simulink library "Lib_Piccolo"  (R2018b)
settings: Solver=VariableStepAuto  StartTime=0.0  StopTime=10.0  RelTol=1e-3
values from neighbouring files (symbols this model uses):
  AccelErrInt2Brakes = 0.15    [SimulationControlConfig16P.m]    (also in SimulationControlConfig16P_LEGACY.m; SimulationControlConfigTAILLESS.m = 0.2; SimulationControlConfigUTAIL.m = 0.2)
  AileronMax = 25    [SimulationControlConfig16P.m]    (also in SimulationControlConfig16P_LEGACY.m; SimulationControlConfigTAILLESS.m; SimulationControlConfigUTAIL.m)
  AileronPower = 0.00268    [SimulationControlConfig16P.m]    (also in SimulationControlConfig16P_LEGACY.m; SimulationControlConfigTAILLESS.m; SimulationControlConfigUTAIL.m)
  AileronSurfaceMax = 45    [SimulationControlConfig16P.m]    (also in SimulationControlConfig16P_LEGACY.m)
  AileronTrim = 0    [SimulationControlConfig16P.m]    (also in SimulationControlConfig16P_LEGACY.m; SimulationControlConfigTAILLESS.m; SimulationControlConfigUTAIL.m)
  Alt = 1000 + TerrainHeight    [SimulationStateConfig.m]
  AltCruise_m = testPlans(testIndx).terrainElevation * 0.3048 + 200    [SimulationControlConfig16P.m]    (also in SimulationControlConfigTAILLESS.m = 1083; SimulationControlConfigUTAIL.m = testPlans(testIndx).terrainElevation * 0.3048 + 152)
  AltitudeRate2PitchCmdIntegratorInit = 0.1    [SimulationControlPre.m]
  AltMax = 10000    [SimulationControlConfig16P.m]    (also in SimulationControlConfig16P_LEGACY.m; SimulationControlConfigTAILLESS.m; SimulationControlConfigUTAIL.m)
  AltMaxAccel = 1.25    [SimulationControlConfig16P.m]    (also in SimulationControlConfig16P_LEGACY.m = 0.9; SimulationControlConfigTAILLESS.m = 1.7; SimulationControlConfigUTAIL.m = 2)
  AltMin = 0    [SimulationControlConfig16P.m]    (also in SimulationControlConfig16P_LEGACY.m; SimulationControlConfigTAILLESS.m; SimulationControlConfigUTAIL.m)
  AltRateCmd2Pitch = 0.50    (= 0.5)    [SimulationControlConfig16P.m]    (also in SimulationControlConfig16P_LEGACY.m = 0.6; SimulationControlConfigTAILLESS.m = 0.2; SimulationControlConfigUTAIL.m = 0.3)
  AltRateError2Pitch = 0.40    (= 0.4)    [SimulationControlConfig16P.m]    (also in SimulationControlConfig16P_LEGACY.m; SimulationControlConfigTAILLESS.m = 0.55; SimulationControlConfigUTAIL.m = 0.55)
  AltRateErrorInt2Pitch = 0.50    (= 0.5)    [SimulationControlConfig16P.m]    (also in SimulationControlConfig16P_LEGACY.m = 0.45; SimulationControlConfigTAILLESS.m; SimulationControlConfigUTAIL.m = 0.75)
  AltRateLpfCutOff = 3    [SimulationControlConfig16P.m]    (also in SimulationControlConfig16P_LEGACY.m; SimulationControlConfigTAILLESS.m = 2; SimulationControlConfigUTAIL.m = 2)
  AutoNosegear2Rudder = 26    [SimulationControlConfig16P.m]    (also in SimulationControlConfig16P_LEGACY.m; SimulationControlConfigTAILLESS.m = 25.2; SimulationControlConfigUTAIL.m = 14)
  b = 5.54    [SimulationControlConfig16P.m]    (also in SimulationControlConfig16P_LEGACY.m; SimulationControlConfigTAILLESS.m = 2.37; SimulationControlConfigUTAIL.m = 2.37)
  Bank2AileronIntegratorInit = 0    [SimulationControlPre.m]
  BankMax_User = BankMax_User/180*pi    (= 0.523598775598)    [SimulationControlConfig16P.m]    (also in SimulationControlConfig16P_LEGACY.m; SimulationControlConfigTAILLESS.m = 0.610865238198; SimulationControlConfigUTAIL.m = 0.628318530718)
  baseLegFlaps = 20    [SimulationControlConfig16P.m]    (also in SimulationControlConfig16P_LEGACY.m = 0; SimulationControlConfigTAILLESS.m = 15; SimulationControlConfigUTAIL.m = 10)
  C = GeneticOpt.C    [SimulationCostFunction.m]
  c = Sw/b    (= 0.841696750903)    [SimulationControlConfig16P.m]    (also in SimulationControlConfig16P_LEGACY.m; SimulationControlConfigTAILLESS.m = 0.354008438819; SimulationControlConfigUTAIL.m = 0.354008438819)
  cell2WheelFactorMG = 5.98    [SimulationSensorConfig16P_LEGACY.m]
  cell2WheelFactorNG = 1    [SimulationSensorConfig16P_LEGACY.m]
  cellSatMaxMG = 15000    [SimulationSensorConfig16P.m]    (also in SimulationSensorConfig16P_LEGACY.m; SimulationSensorConfigTAILLESS7P.m; SimulationSensorConfigUTAIL7P.m)
  cellSatMaxNG = 1000    [SimulationSensorConfig16P.m]    (also in SimulationSensorConfig16P_LEGACY.m; SimulationSensorConfigTAILLESS7P.m; SimulationSensorConfigUTAIL7P.m)
  cellSatMinMG = -15000    [SimulationSensorConfig16P.m]    (also in SimulationSensorConfig16P_LEGACY.m; SimulationSensorConfigTAILLESS7P.m; SimulationSensorConfigUTAIL7P.m)
  cellSatMinNG = -1000    [SimulationSensorConfig16P.m]    (also in SimulationSensorConfig16P_LEGACY.m; SimulationSensorConfigTAILLESS7P.m; SimulationSensorConfigUTAIL7P.m)
  CL_Limit = CL_Max    (= 0.54)    [SimulationControlConfig16P.m]    (also in SimulationControlConfig16P_LEGACY.m; SimulationControlConfigTAILLESS.m; SimulationControlConfigUTAIL.m = 0.53)
  CL_Max = 0.54    [SimulationControlConfig16P.m]    (also in SimulationControlConfig16P_LEGACY.m; SimulationControlConfigTAILLESS.m; SimulationControlConfigUTAIL.m = 0.53)
  CL_Max_Nom = 0.465    [SimulationControlConfig16P.m]    (also in SimulationControlConfig16P_LEGACY.m; SimulationControlConfigTAILLESS.m = 0.39; SimulationControlConfigUTAIL.m)
  CL_Min = 0    [SimulationControlConfig16P.m]    (also in SimulationControlConfig16P_LEGACY.m; SimulationControlConfigTAILLESS.m; SimulationControlConfigUTAIL.m)
  ClimbMaxFraction = 0.35    [SimulationControlConfig16P.m]    (also in SimulationControlConfig16P_LEGACY.m = 0.24; SimulationControlConfigTAILLESS.m = 0.19; SimulationControlConfigUTAIL.m = 0.21)
  ClimboutMaxBank = 7.0    (= 7)    [SimulationControlConfig16P.m]    (also in SimulationControlConfig16P_LEGACY.m; SimulationControlConfigTAILLESS.m = 5; SimulationControlConfigUTAIL.m)
  ClimboutTimer = 7.0    (= 7)    [SimulationControlConfig16P.m]    (also in SimulationControlConfig16P_LEGACY.m; SimulationControlConfigTAILLESS.m; SimulationControlConfigUTAIL.m)
  dCl_per_dFlap = 0.005581818    [SimulationControlConfig16P.m]    (also in SimulationControlConfig16P_LEGACY.m = 0; SimulationControlConfigTAILLESS.m = 0; SimulationControlConfigUTAIL.m = 0)
  DecelerationCmd = 3.1    [SimulationControlConfig16P.m]    (also in SimulationControlConfig16P_LEGACY.m; SimulationControlConfigTAILLESS.m = 0.1; SimulationControlConfigUTAIL.m = 0.1)
  DeRotateLogicEndTimer = abs((NoseDownLimit_Deg-1)/DeRotateRamp_Dps)    [SimulationControlConfig16P.m]    (also in SimulationControlConfig16P_LEGACY.m; SimulationControlConfigTAILLESS.m; SimulationControlConfigUTAIL.m)
  DeRotateLogicHoldNoseUpTimer = 0.1    [SimulationControlConfig16P.m]    (also in SimulationControlConfig16P_LEGACY.m; SimulationControlConfigTAILLESS.m; SimulationControlConfigUTAIL.m)
  DeRotateLogicTimerTimeout = 2    [SimulationControlConfig16P.m]    (also in SimulationControlConfig16P_LEGACY.m; SimulationControlConfigTAILLESS.m; SimulationControlConfigUTAIL.m)
  DeRotateLowerCmdSaturation = 0    [SimulationControlConfig16P.m]    (also in SimulationControlConfig16P_LEGACY.m; SimulationControlConfigTAILLESS.m; SimulationControlConfigUTAIL.m)
  DeRotateRamp_Dps = 3    [SimulationControlConfig16P.m]    (also in SimulationControlConfig16P_LEGACY.m; SimulationControlConfigTAILLESS.m = 8; SimulationControlConfigUTAIL.m = 8)
  DeRotateUpperCmdSaturation = 7    [SimulationControlConfig16P.m]    (also in SimulationControlConfig16P_LEGACY.m; SimulationControlConfigTAILLESS.m; SimulationControlConfigUTAIL.m)
  DescentMaxFraction = 0.22    [SimulationControlConfig16P.m]    (also in SimulationControlConfig16P_LEGACY.m = 0.2; SimulationControlConfigTAILLESS.m = 0.17; SimulationControlConfigUTAIL.m = 0.17)
  DesktopSimTerrainOffset_m = 0.406    [SimulationAircraftConfig.m]
  downwindFlaps = 0    [SimulationControlConfig16P.m]    (also in SimulationControlConfig16P_LEGACY.m; SimulationControlConfigTAILLESS.m; SimulationControlConfigUTAIL.m)
  DP_init = 0.5*1.225*V_init^2    [SimulationControlConfig16P.m]    (also in SimulationControlConfig16P_LEGACY.m; SimulationControlConfigTAILLESS.m; SimulationControlConfigUTAIL.m)
  dscNoiseMG = 1    [SimulationSensorConfig16P_LEGACY.m]
  dscNoiseNG = 0.25    [SimulationSensorConfig16P_LEGACY.m]
  DSCnumBits = 24    [SimulationSensorConfig16P.m]    (also in SimulationSensorConfig16P_LEGACY.m; SimulationSensorConfigTAILLESS7P.m; SimulationSensorConfigUTAIL7P.m)
  DSCRangeMaxMG = 15000    [SimulationSensorConfig16P.m]    (also in SimulationSensorConfig16P_LEGACY.m; SimulationSensorConfigTAILLESS7P.m; SimulationSensorConfigUTAIL7P.m)
  DSCRangeMaxNG = 1000    [SimulationSensorConfig16P.m]    (also in SimulationSensorConfig16P_LEGACY.m; SimulationSensorConfigTAILLESS7P.m; SimulationSensorConfigUTAIL7P.m)
  DSCRangeMinMG = -15000    [SimulationSensorConfig16P.m]    (also in SimulationSensorConfig16P_LEGACY.m; SimulationSensorConfigTAILLESS7P.m; SimulationSensorConfigUTAIL7P.m)
  DSCRangeMinNG = -1000    [SimulationSensorConfig16P.m]    (also in SimulationSensorConfig16P_LEGACY.m; SimulationSensorConfigTAILLESS7P.m; SimulationSensorConfigUTAIL7P.m)
  dt = DLLSim.dt    [SimulationTimeStep.m]    (also in SimulationTrim.m = 0.02)
  EarlyTouchdownThreshold = 3.0    (= 3)    [SimulationControlConfig16P.m]    (also in SimulationControlConfig16P_LEGACY.m; SimulationControlConfigTAILLESS.m = 2.2; SimulationControlConfigUTAIL.m = 2.5)
  ElevatorDeflectionRate = 15    [SimulationControlConfig16P.m]    (also in SimulationControlConfig16P_LEGACY.m = 12; SimulationControlConfigTAILLESS.m = 10; SimulationControlConfigUTAIL.m = 12)
  ElevatorMax = 25    [SimulationControlConfig16P.m]    (also in SimulationControlConfig16P_LEGACY.m; SimulationControlConfigTAILLESS.m; SimulationControlConfigUTAIL.m)
  ElevatorPower = -0.002209    [SimulationControlConfig16P.m]    (also in SimulationControlConfig16P_LEGACY.m; SimulationControlConfigTAILLESS.m = -0.002956; SimulationControlConfigUTAIL.m = -0.00205983)
  ElevatorTrim = -3.5    [SimulationControlConfig16P.m]    (also in SimulationControlConfig16P_LEGACY.m; SimulationControlConfigTAILLESS.m = -6; SimulationControlConfigUTAIL.m = -8)
  elevonBias = 0    [SimulationControlConfig16P.m]    (also in SimulationControlConfig16P_LEGACY.m; SimulationControlConfigTAILLESS.m; SimulationControlConfigUTAIL.m)
  Enable_TAS_Protection = 0    [SimulationControlConfig16P.m]    (also in SimulationControlConfig16P_LEGACY.m; SimulationControlConfigTAILLESS.m; SimulationControlConfigUTAIL.m)
  EnableCrossTrackAbort = 1    [SimulationControlConfig16P.m]    (also in SimulationControlConfigTAILLESS.m; SimulationControlConfigUTAIL.m)
  EnergyBandwidth = 0.02    [SimulationControlConfig16P.m]    (also in SimulationControlConfig16P_LEGACY.m; SimulationControlConfigTAILLESS.m = 0.06; SimulationControlConfigUTAIL.m = 0.06)
  EngineLhFuelCut = 0    [SimulationAircraftConfig.m]
  EngineRhFuelCut = 0    [SimulationAircraftConfig.m]
  FastThrottleRate = 0.075    [SimulationControlConfig16P.m]    (also in SimulationControlConfig16P_LEGACY.m = 0.05; SimulationControlConfigTAILLESS.m = 0.1; SimulationControlConfigUTAIL.m = 0.1)
  FilterWarmUpTime = 2    [SimulationSensorConfig16P.m]    (also in SimulationSensorConfig16P_LEGACY.m; SimulationSensorConfigTAILLESS7P.m; SimulationSensorConfigUTAIL7P.m)
  finalApproachFlaps = 20    [SimulationControlConfig16P.m]    (also in SimulationControlConfig16P_LEGACY.m = 0; SimulationControlConfigTAILLESS.m = 22; SimulationControlConfigUTAIL.m = 10)
  FinalDescentSlope_Deg = testPlans(testIndx).descentSlope    [SimulationControlConfig16P.m]    (also in SimulationControlConfig16P_LEGACY.m; SimulationControlConfigTAILLESS.m; SimulationControlConfigUTAIL.m)
  flapMax = 0    [SimulationControlConfig16P.m]    (also in SimulationControlConfig16P_LEGACY.m; SimulationControlConfigTAILLESS.m; SimulationControlConfigUTAIL.m)
  flapRate = 7.5    [SimulationControlConfig16P.m]    (also in SimulationControlConfig16P_LEGACY.m; SimulationControlConfigTAILLESS.m = 6.6; SimulationControlConfigUTAIL.m)
  FlareHeight = 5    [SimulationControlConfig16P.m]    (also in SimulationControlConfig16P_LEGACY.m = 4.8; SimulationControlConfigTAILLESS.m = 2.5; SimulationControlConfigUTAIL.m = 2)
  FlareVerticalRate_mps = -0.4    [SimulationControlConfig16P.m]    (also in SimulationControlConfig16P_LEGACY.m = -0.5; SimulationControlConfigTAILLESS.m = -0.15; SimulationControlConfigUTAIL.m = -0.15)
  Fp_Aileron = 0.55*2*pi*RollRateLpfCutoff*dt    [SimulationControlConfig16P.m]    (also in SimulationControlConfig16P_LEGACY.m; SimulationControlConfigTAILLESS.m; SimulationControlConfigUTAIL.m)
  Fp_Alt = 0.55*AltBandwidth    (= 0.099)    [SimulationControlConfig16P.m]    (also in SimulationControlConfig16P_LEGACY.m; SimulationControlConfigTAILLESS.m = 0.587477826221; SimulationControlConfigUTAIL.m = 0.69115038379)
  Fp_AltRate = 0.55*2*pi*AltRateLpfCutOff*dt    [SimulationControlConfig16P.m]    (also in SimulationControlConfig16P_LEGACY.m; SimulationControlConfigTAILLESS.m; SimulationControlConfigUTAIL.m)
  Fp_Elevator = 0.55*2*pi*PitchRateLpfCutoff*dt    [SimulationControlConfig16P.m]    (also in SimulationControlConfig16P_LEGACY.m; SimulationControlConfigTAILLESS.m; SimulationControlConfigUTAIL.m)
  Fp_Energy = 0.55*2*pi*EnergyBandwidth    (= 0.069115038379)    [SimulationControlConfig16P.m]    (also in SimulationControlConfig16P_LEGACY.m; SimulationControlConfigTAILLESS.m = 0.207345115137; SimulationControlConfigUTAIL.m = 0.207345115137)
  Fp_Energy2 = 0.55*2*pi*EnergyBandwidth*dt    [SimulationControlConfig16P.m]    (also in SimulationControlConfig16P_LEGACY.m; SimulationControlConfigTAILLESS.m; SimulationControlConfigUTAIL.m)
  Fp_Pitch = 0.55*2*pi*PitchBandwidth    (= 2.76460153516)    [SimulationControlConfig16P.m]    (also in SimulationControlConfig16P_LEGACY.m = 3.11017672705; SimulationControlConfigTAILLESS.m = 3.80132711084; SimulationControlConfigUTAIL.m = 2.41902634326)
  Fp_Pitch_2 = 0.55*2*pi*PitchBandwidth*dt    [SimulationControlConfig16P.m]    (also in SimulationControlConfig16P_LEGACY.m; SimulationControlConfigTAILLESS.m; SimulationControlConfigUTAIL.m)
  Fp_Roll = RollBandwidth^2    (= 1)    [SimulationControlConfig16P.m]    (also in SimulationControlConfig16P_LEGACY.m = 1.44; SimulationControlConfigTAILLESS.m; SimulationControlConfigUTAIL.m)
  Fp_Rudder = 0.55*2*pi*YawRateLpfCutoff*dt    [SimulationControlConfig16P.m]    (also in SimulationControlConfig16P_LEGACY.m; SimulationControlConfigTAILLESS.m; SimulationControlConfigUTAIL.m)
  Fp_TAS = 0.55*2*pi*TASBandwidth    (= 0.103672557568)    [SimulationControlConfig16P.m]    (also in SimulationControlConfig16P_LEGACY.m; SimulationControlConfigTAILLESS.m = 0.172787595947; SimulationControlConfigUTAIL.m = 0.172787595947)
  Fp_TAS_Filter = 2*pi*TasLpfCutoff*dt    [SimulationControlConfig16P.m]    (also in SimulationControlConfig16P_LEGACY.m; SimulationControlConfigTAILLESS.m; SimulationControlConfigUTAIL.m)
  Fp_Turn = 0.55*2*pi*TurnErrLPFcutoff    (= 0.0345575191895)    [SimulationControlConfig16P.m]    (also in SimulationControlConfig16P_LEGACY.m; SimulationControlConfigTAILLESS.m = 0.172787595947; SimulationControlConfigUTAIL.m = 0.172787595947)
  Fp_TurnDerr = 0.55*2*pi*TurnDerivativeLPFcutoff    (= 0.0345575191895)    [SimulationControlConfig16P.m]    (also in SimulationControlConfig16P_LEGACY.m; SimulationControlConfigTAILLESS.m = 0.172787595947; SimulationControlConfigUTAIL.m = 0.172787595947)
  FTV = 3    [SimulationAircraftConfig.m]
  ftvStaticPositionError = 1/1.18    (= 0.847457627119)    [SimulationSensorConfig16P.m]    (also in SimulationSensorConfig16P_LEGACY.m; SimulationSensorConfigTAILLESS7P.m = 1; SimulationSensorConfigUTAIL7P.m = 1)
  g = 9.81    [SimulationStateConfig.m]
  GustSpd_Kts = testPlans(testIndx).gustSpd    [SimulationStateConfig.m]
  GustTriggerVal = testPlans(testIndx).gustTriggerVal    [SimulationStateConfig.m]
  HeadingErr2TurnRate = 0.5    [SimulationControlConfig16P.m]    (also in SimulationControlConfig16P_LEGACY.m; SimulationControlConfigTAILLESS.m; SimulationControlConfigUTAIL.m)
  HeadingErrDer2TurnRate = 0.3    [SimulationControlConfig16P.m]    (also in SimulationControlConfig16P_LEGACY.m; SimulationControlConfigTAILLESS.m; SimulationControlConfigUTAIL.m)
  IASbounce = IASstall*0.8    [SimulationControlPre.m]
  IAScruiseCMD = sqrt(2*m*9.81/(1.225*Sw*CL_cruise))    [SimulationControlConfig16P.m]    (also in SimulationControlConfig16P_LEGACY.m; SimulationControlConfigTAILLESS.m; SimulationControlConfigUTAIL.m)
  IASfinalCMD = 1.12 * IASmin    [SimulationControlConfig16P.m]    (also in SimulationControlConfig16P_LEGACY.m = 1.10 * IASmin; SimulationControlConfigTAILLESS.m = 1.10 * IASmin; SimulationControlConfigUTAIL.m = 1.15 * IASmin)
  IASflareCMD = IASstall    [SimulationControlConfig16P.m]    (also in SimulationControlConfig16P_LEGACY.m; SimulationControlConfigTAILLESS.m; SimulationControlConfigUTAIL.m)
  IASmax = 64    [SimulationControlConfig16P.m]    (also in SimulationControlConfig16P_LEGACY.m = 46; SimulationControlConfigTAILLESS.m = 38.58; SimulationControlConfigUTAIL.m = 35)
  IASmin = sqrt(2*m*9.81/(1.225*Sw*0.9*CL_Max_Nom))    [SimulationControlConfig16P.m]    (also in SimulationControlConfig16P_LEGACY.m; SimulationControlConfigTAILLESS.m; SimulationControlConfigUTAIL.m)
  IASshortCMD = IASstall    [SimulationControlConfig16P.m]    (also in SimulationControlConfig16P_LEGACY.m; SimulationControlConfigTAILLESS.m; SimulationControlConfigUTAIL.m)
  IASstall = sqrt(2*m*9.81/(1.225*Sw*CL_Max))    [SimulationControlConfig16P.m]    (also in SimulationControlConfig16P_LEGACY.m; SimulationControlConfigTAILLESS.m; SimulationControlConfigUTAIL.m)
  inFlight = 1    [SimulationControlConfig16P.m]    (also in SimulationControlConfigTAILLESS.m; SimulationControlConfigUTAIL.m)
  JetCatOffset = 5    [SimulationControlConfig16P.m]    (also in SimulationControlConfig16P_LEGACY.m)
  LaunchRollingElevator = -1.5    [SimulationControlConfig16P.m]    (also in SimulationControlConfig16P_LEGACY.m; SimulationControlConfigTAILLESS.m = 1; SimulationControlConfigUTAIL.m = 1)
  ldg_NosegearMax = 10    [SimulationControlConfig16P.m]    (also in SimulationControlConfig16P_LEGACY.m; SimulationControlConfigTAILLESS.m; SimulationControlConfigUTAIL.m)
  ldg_TrackVyErrInt2Nosegear = 0.1250    (= 0.125)    [SimulationControlConfig16P.m]    (also in SimulationControlConfig16P_LEGACY.m; SimulationControlConfigTAILLESS.m = 0.00714285714286; SimulationControlConfigUTAIL.m = 0.00714285714286)
  ldg_TrackVyErrPro2Nosegear = 0.35    [SimulationControlConfig16P.m]    (also in SimulationControlConfig16P_LEGACY.m; SimulationControlConfigTAILLESS.m = 0.0546666666667; SimulationControlConfigUTAIL.m = 0.0546666666667)
  ldg_TrackY2Vy = 0.07    [SimulationControlConfig16P.m]    (also in SimulationControlConfig16P_LEGACY.m; SimulationControlConfigTAILLESS.m = 0.17; SimulationControlConfigUTAIL.m = 0.17)
  ldg_Vy2NosegearScalingPower = 1.075    [SimulationControlConfig16P.m]    (also in SimulationControlConfig16P_LEGACY.m; SimulationControlConfigTAILLESS.m = 0.6; SimulationControlConfigUTAIL.m = 0.5)
  ldg_Y2VyScalingPower = 0.175    [SimulationControlConfig16P.m]    (also in SimulationControlConfig16P_LEGACY.m; SimulationControlConfigTAILLESS.m = 0; SimulationControlConfigUTAIL.m = 0)
  ldg_YawRate2Nosegear = 0.175    [SimulationControlConfig16P.m]    (also in SimulationControlConfig16P_LEGACY.m; SimulationControlConfigTAILLESS.m = 0.065; SimulationControlConfigUTAIL.m = 0.065)
  LiftSlope = 0.064285    [SimulationControlConfig16P.m]    (also in SimulationControlConfig16P_LEGACY.m; SimulationControlConfigTAILLESS.m = 0.058631; SimulationControlConfigUTAIL.m)
  LPFaileronInit = 0    [SimulationControlPre.m]
  LPFclestInit = 0    [SimulationControlPre.m]
  LPFenergyFFInit = 0    [SimulationControlPre.m]
  LPFtasInit = V_init + 2    [SimulationControlPre.m]
  LPFthrottleInit = ThrottleTrim    [SimulationControlPre.m]
  LPFturnErrInit = 0    [SimulationControlPre.m]
  ... (+115 more)
undefined symbols (not defined in the file or in its folder): abortFlag, alphaHPF, apmDelay, BRWNOUT, CRAWOR, CRAWUR, DiscIntNeverNeededParam, DLLSim, DLLSimStep, ECOMOR, ECOMUR, Fp_Tas, GustTrigger_HeightAgl_m, IPSTAT, LCINTEG, Ldg_Persist_Time, LOWER_FLAGS, MSG_ENABLE, NoiseStd, OLDVAL, OVERRIDE_ENABLE, OVERRIDE_VALUE, REBOOT, reversionEnable, revIASMax, revIASMin, revPitchMax, revPitchMin, revPitchRateMax, revRollMax, revRollRateMax, SAMPLE, SCALON, SensorModel, sigbuilder_block, Sim_Vx, Sim_Vy, Sim_Vz, Sim_Xpos, Sim_Ypos, Sim_Zpos, SYSOR, SYSUR, TARE, TEMPOR, TEMPUR, testIndx, testPlan, testPlans, Trim_piccoloInCmd, Trim_REFSI_FD_IN_nmodeCgShifterCmd_Ft, Trim_REFSI_FD_IN_nmodeFlapLhIBCmd_Deg, Trim_REFSI_FD_IN_nmodeFlapLhOBCmd_Deg, Trim_REFSI_FD_IN_nmodeFlapRhIBCmd_Deg, Trim_REFSI_FD_IN_nmodeFlapRhOBCmd_Deg, Trim_REFSI_FD_IN_nmodeSlatLhCmd_Deg, Trim_REFSI_FD_IN_nmodeSlatRhCmd_Deg, Trim_REFSI_FD_IN_nmodeSplrLhInbdCmd_Deg, Trim_REFSI_FD_IN_nmodeSplrLhOutbdCmd_Deg ... (+5)
libraries: simulink x866, aerolibconvert2 x60, $bdroot x52, aerolibatmos2 x5, dspswit3 x5, simulink_extras x4, dsparch4 x2, Lib_Piccolo_Alt x2, eeGeneralControl x1, dspindex x1
(part 4 of 44)

== system Lib_Piccolo/IAS Min Calc ==
  Compare To Constant : simulink/Logic and Bit Operations/Compare To Constant  relop=<  const=10  OutDataTypeStr=boolean
  Constant : Constant  Value=(2*m*g)
  Constant1 : Constant  Value=CL_Max
  Constant2 : Constant  Value=CL_Max_Nom
  Constant3 : Constant  Value=(2*m*g)
  Divide : Product  Inputs=*/
  Divide1 : Product  Inputs=*/
  Gain : Gain  Gain=dCl_per_dFlap
  Gain1 : Gain  Gain=1.225*Sw*0.9
  Gain2 : Gain  Gain=1.225*Sw
  Sqrt : Sqrt  SaturateOnIntegerOverflow=on
  Sqrt1 : Sqrt  SaturateOnIntegerOverflow=on
  Sum : Sum  Inputs=|++
  Sum1 : Sum  Inputs=++|
  Switch : Switch  Criteria=u2 > Threshold  Threshold=0.5
  Terminator : Terminator
  IASmin : Outport
  tag scope: IASmin=global, IASstall=global
  wires:
  Sqrt/1 -> Switch/1, [IASmin]  "Sim.IASmin"
  Constant/1 -> Divide/1
  Constant2/1 -> Sum/1
  [flapCmd] -> Gain/1
  Gain/1 -> Sum1/1, Sum/2
  Sum/1 -> Gain1/1
  Gain1/1 -> Divide/2
  Divide/1 -> Sqrt/1
  Constant1/1 -> Sum1/2
  Sum1/1 -> Gain2/1
  Gain2/1 -> Divide1/2
  Constant3/1 -> Divide1/1
  Divide1/1 -> Sqrt1/1
  Sqrt1/1 -> Switch/3, Terminator/1, [IASstall]  "Sim.IASstall"
  Switch/1 -> IASmin/1  "Sim.IASminAP"
  [Pic_AP_Mode] -> Compare To Constant/1
  Compare To Constant/1 -> Switch/2

== system Lib_Piccolo/LDG TAS Cmd ==
  note: Check if in Short Final
  note: Check if in Flare
  Feedback Bus : Inport
  Bus Selector : BusSelector  OutputSignals=apMode
  Bus Selector1 : BusSelector  OutputSignals=apMode
  CAS2TAS : Subsystem
  Compare To Constant1 : simulink/Logic and Bit Operations/Compare To Constant  relop=>=  const=10  OutDataTypeStr=boolean
  Compare To Constant4 : simulink/Logic and Bit Operations/Compare To Constant  relop=>=  const=9  OutDataTypeStr=boolean
  Constant : Constant  Value=IASmax
  Constant2 : Constant  Value=IASshortCMD+testPlans(testIndx).speedOffset
  Constant3 : Constant  Value=IASfinalCMD+testPlans(testIndx).speedOffset
  Constant4 : Constant  Value=IASflareCMD
  IAS Min Calc : $bdroot/IAS Min Calc  SystemSampleTime=-1
  Multiply : Product
  NOT : Logic  Operator=NOT  IconShape=distinctive  AllPortsSameDT=off  OutDataTypeStr=boolean
  NOT1 : Logic  Operator=NOT  IconShape=distinctive  AllPortsSameDT=off  OutDataTypeStr=boolean
  Saturation Dynamic : simulink/Discontinuities/Saturation Dynamic  OutMin=[]  OutMax=[]  OutDataTypeStr=Inherit: Same as second input  OutDataType=fixdt(1, 16)  OutScaling=2^-10  DoSatur=off
  Switch1 : Switch  Criteria=u2 > Threshold
  Switch2 : Switch  Criteria=u2 > Threshold
  Sim.TAScmd : Outport
  tag scope: Sim_TAScmd=global
  wires:
  CAS2TAS/1(Out1) -> Multiply/2
  Switch2/1 -> Saturation Dynamic/2
  Constant2/1 -> Switch2/3
  Constant4/1 -> Switch1/3
  Constant3/1 -> Switch2/1
  Switch1/1 -> Multiply/1  "Sim.IAScmd"
  Multiply/1 -> [Sim_TAScmd], Sim.TAScmd/1  "Sim.TAScmd"
  Compare To Constant4/1 -> NOT/1
  Bus Selector/1 -> Compare To Constant4/1  "<apMode>"
  NOT/1 -> Switch2/2
  Feedback Bus/1 -> Bus Selector1/1, Bus Selector/1, CAS2TAS/1(In1)
  Bus Selector1/1 -> Compare To Constant1/1  "<apMode>"
  Compare To Constant1/1 -> NOT1/1
  NOT1/1 -> Switch1/2
  IAS Min Calc/1 -> Saturation Dynamic/3
  Constant/1 -> Saturation Dynamic/1
  Saturation Dynamic/1 -> Switch1/1

== system Lib_Piccolo/LDG TAS Cmd No Offset ==
  note: Check if in Short Final
  note: Check if in Flare
  Feedback Bus : Inport
  Bus Selector : BusSelector  OutputSignals=apMode
  Bus Selector1 : BusSelector  OutputSignals=apMode
  CAS2TAS : Subsystem
  Compare To Constant1 : simulink/Logic and Bit Operations/Compare To Constant  relop=>=  const=10  OutDataTypeStr=boolean
  Compare To Constant4 : simulink/Logic and Bit Operations/Compare To Constant  relop=>=  const=9  OutDataTypeStr=boolean
  Constant : Constant  Value=IASmax
  Constant2 : Constant  Value=IASshortCMD
  Constant3 : Constant  Value=IASfinalCMD
  Constant4 : Constant  Value=IASflareCMD
  IAS Min Calc : $bdroot/IAS Min Calc  SystemSampleTime=-1
  Multiply : Product
  NOT : Logic  Operator=NOT  IconShape=distinctive  AllPortsSameDT=off  OutDataTypeStr=boolean
  NOT1 : Logic  Operator=NOT  IconShape=distinctive  AllPortsSameDT=off  OutDataTypeStr=boolean
  Saturation Dynamic : simulink/Discontinuities/Saturation Dynamic  OutMin=[]  OutMax=[]  OutDataTypeStr=Inherit: Same as second input  OutDataType=fixdt(1, 16)  OutScaling=2^-10  DoSatur=off
  Switch1 : Switch  Criteria=u2 > Threshold
  Switch2 : Switch  Criteria=u2 > Threshold
  Sim.TAScmd : Outport
  tag scope: Sim_TAScmd=global
  wires:
  CAS2TAS/1(Out1) -> Multiply/2
  Switch2/1 -> Saturation Dynamic/2
  Constant2/1 -> Switch2/3
  Constant4/1 -> Switch1/3
  Constant3/1 -> Switch2/1
  Switch1/1 -> Multiply/1  "Sim.IAScmd"
  Multiply/1 -> [Sim_TAScmd], Sim.TAScmd/1  "Sim.TAScmd"
  Compare To Constant4/1 -> NOT/1
  Bus Selector/1 -> Compare To Constant4/1  "<apMode>"
  NOT/1 -> Switch2/2
  Feedback Bus/1 -> Bus Selector1/1, Bus Selector/1, CAS2TAS/1(In1)
  Bus Selector1/1 -> Compare To Constant1/1  "<apMode>"
  Compare To Constant1/1 -> NOT1/1
  NOT1/1 -> Switch1/2
  IAS Min Calc/1 -> Saturation Dynamic/3
  Constant/1 -> Saturation Dynamic/1
  Saturation Dynamic/1 -> Switch1/1

== system Lib_Piccolo/Latch ==
  D : Inport
  Enable/!Rst : Inport  Port=2
  AND : Logic  IconShape=distinctive  AllPortsSameDT=off  OutDataTypeStr=boolean
  Constant : Constant
  OR : Logic  Operator=OR  IconShape=distinctive  AllPortsSameDT=off  OutDataTypeStr=boolean
  Switch : Switch  Criteria=u2 > Threshold  Threshold=0.5
  Unit Delay : UnitDelay  SampleTime=-1
  Q_Latched : Outport
  wires:
  Unit Delay/1 -> OR/2
  Switch/1 -> Q_Latched/1, Unit Delay/1
  D/1 -> Switch/3, OR/1
  OR/1 -> AND/1
  AND/1 -> Switch/2
  Enable/!Rst/1 -> AND/2
  Constant/1 -> Switch/1

== system Lib_Piccolo/Pic Airspeed Model ==
  note: $\rho = \frac{P\cdot MW}{R\cdot T}$
  note: $IAS = \sqrt{\frac{2\cdot P_{dynamic}}{\rho_0}}$
  note: $P_{dynamic} = P_{dynamic\_sensor} \cdot Correction$
  note: $P_{static} = P_{static} + P_{dynamic\_sensor} - P_{dynamic}$
  note: $TAS = \frac{IAS}{\sqrt{\frac{\rho}{\rho_0}}}$
  OAT_C : Inport
  Static_Pa : Inport  Port=2
  Dynamic_Pa : Inport  Port=3
  Constant : Constant  Value=0
  Constant1 : Constant  Value=0
  Divide{,1..3} (4 alike) : Product  Inputs=*/
  Gain : Gain  Gain=2
  Gain1 : Gain  Gain=correction
  Ideal Gas Constant : Gain  Gain=8.314463
  Kelvin Offset : Constant  Value=273.15
  MW (kg/mol) : Gain  Gain=28.9647/1000
  Max : MinMax  Function=max  Inputs=2
  Max1 : MinMax  Function=max  Inputs=2
  Sqrt : Sqrt  SaturateOnIntegerOverflow=on
  Sqrt1 : Sqrt  SaturateOnIntegerOverflow=on
  Sum : Sum  Inputs=++|
  Sum1 : Sum  Inputs=-++
  rho SL ISA : Constant  Value=1.225
  TAS : Outport
  IAS : Outport  Port=2
  Sim.PicDensity_kg/m3 : Outport  Port=3
  wires:
  OAT_C/1 -> Sum/2
  Kelvin Offset/1 -> Sum/1
  Sum/1 -> Ideal Gas Constant/1
  MW (kg/mol)/1 -> Divide/1
  Ideal Gas Constant/1 -> Divide/2
  Divide/1 -> Sim.PicDensity_kg/m3/1, Divide2/1  "IdealDensity_kg/m3"
  Gain1/1 -> Sum1/1, Gain/1  "Pdynamic"
  Gain/1 -> Divide1/1
  Divide1/1 -> Max/1
  rho SL ISA/1 -> Divide2/2, Divide1/2
  Divide2/1 -> Max1/1
  Divide3/1 -> TAS/1  "Sim.Pic_TAS"
  Sqrt/1 -> IAS/1, Divide3/1  "Sim.Pic_IAS"
  Dynamic_Pa/1 -> Sum1/2, Gain1/1  "Pdynamic_sensor"
  Sum1/1 -> MW (kg/mol)/1  "Pstatic"
  Sqrt1/1 -> Divide3/2
  Static_Pa/1 -> Sum1/3
  Max/1 -> Sqrt/1
  Constant/1 -> Max/2
  Constant1/1 -> Max1/2
  Max1/1 -> Sqrt1/1

== system Lib_Piccolo/Piccolo State Machine ==
  SimOutBus In : Inport
  In1 : Inport  Port=2
  Bus Assignment : BusAssignment  AssignedSignals=apMode
  Bus Selector : BusSelector  OutputSignals=apMode,IAS_mps,Sim_VGround
  Constant4 : Constant  Value=inFlight
  Flight State Machine : Subsystem
  Landing State Machine : Subsystem
  Switch4 : Switch  Threshold=1
  SimOutBus Out : Outport
  Out1 : Outport  Port=2
  tag scope: Pic_AP_Mode=global
  wires:
  Bus Selector/3 -> Flight State Machine/3(GroundSpeed)  "<Sim_VGround>"
  In1/1 -> Bus Assignment/1, Bus Selector/1
  Bus Assignment/1 -> Out1/1
  SimOutBus In/1 -> SimOutBus Out/1
  Constant4/1 -> Switch4/2  "inFlight"
  Bus Selector/1 -> Flight State Machine/1(<apMode>), Landing State Machine/1(<apMode>)  "<apMode>"
  Landing State Machine/1(Sim.apMode) -> Switch4/3
  Flight State Machine/1(Sim.apMode) -> Switch4/1
  Switch4/1 -> [Pic_AP_Mode], Bus Assignment/2  "Sim.apMode"
  Bus Selector/2 -> Flight State Machine/2(IAS)  "<IAS_mps>"

== system Lib_Piccolo/Piccolo State Machine FLIGHT LEGACY ==
  note: Assume maneuvers performed in 'Flying' State
  note: Moved to Vertical Track Following Guidance in Next Block
  SimOutBus In : Inport
  In1 : Inport  Port=2
  Bus Assignment : BusAssignment  AssignedSignals=apMode
  Constant : Constant  Value=4  OutDataTypeStr=uint8
  Flare Detection : Subsystem
  ShortFinal Detection : Subsystem  Commented=on
  SimOutBus Out : Outport
  Out1 : Outport  Port=2
  tag scope: Pic_AP_Mode=global
  wires:
  In1/1 -> Bus Assignment/1
  Constant/1 -> Bus Assignment/2, [Pic_AP_Mode]  "Sim.apMode"
  Bus Assignment/1 -> Out1/1
  SimOutBus In/1 -> SimOutBus Out/1

== system Lib_Piccolo/Piccolo State Machine LDG ==
  note: Moved to Vertical Track Following Guidance in Next Block
  SimOutBus In : Inport
  In1 : Inport  Port=2
  Bus Assignment : BusAssignment  AssignedSignals=apMode
  Bus Selector : BusSelector  OutputSignals=apMode
  Compare To Constant1 : simulink/Logic and Bit Operations/Compare To Constant  relop=>  const=0  OutDataTypeStr=boolean
  Constant : Constant  Value=9
  Constant1 : Constant  Value=10
  Constant2 : Constant  Value=11
  Constant3 : Constant  Value=8
  Data Type Conversion : DataTypeConversion  OutDataTypeStr=uint8
  Flare Detection : Subsystem
  FlareLatch : Subsystem
  NOT : Logic  Operator=NOT  IconShape=distinctive  AllPortsSameDT=off  OutDataTypeStr=boolean
  NOT1 : Logic  Operator=NOT  IconShape=distinctive  AllPortsSameDT=off  OutDataTypeStr=boolean
  ShortFinal Detection : Subsystem  Commented=on
  Switch{,1..3} (4 alike) : Switch  Criteria=u2 > Threshold
  SimOutBus Out : Outport
  Out1 : Outport  Port=2
  tag scope: Pic_AP_Mode=global
  wires:
  In1/1 -> Bus Assignment/1, Bus Selector/1
  [ShortFinalFlag] -> Compare To Constant1/1
  Constant/1 -> Switch/3
  Switch/1 -> Switch1/1
  Constant1/1 -> Switch1/3
  Switch1/1 -> Switch2/1
  Constant2/1 -> Switch2/3
  Switch2/1 -> Data Type Conversion/1, [Pic_AP_Mode]  "Sim.apMode"
  Bus Selector/1 -> Switch3/1  "<apMode>"
  Bus Assignment/1 -> Out1/1
  Compare To Constant1/1 -> Switch/2
  SimOutBus In/1 -> SimOutBus Out/1
  Switch3/1 -> Switch/1
  [FinalFlag] -> NOT1/1
  Constant3/1 -> Switch3/3
  NOT1/1 -> Switch3/2
  [FlareFlag] -> FlareLatch/2(FlareFlag)
  FlareLatch/1(FlareLatch) -> Switch1/2
  [Pic_AP_Mode] -> FlareLatch/1(apMode)
  NOT/1 -> Switch2/2
  [TouchdownDetectedFlag] -> NOT/1
  Data Type Conversion/1 -> Bus Assignment/2

== system Lib_Piccolo/Pitch to Elevator ==
  note: Euler to Body Conversion, Reference Signal Generation
  note: Scalar Saturation
  note: Output Filtering, Ramp & Reversion Logic
  note: Dynamic Inversion Components
  note: P I Components
  note: Damp and STIFF are non-dimentional;
      | CP has the unit of 1/deg
  PitchCmd_Euler : Inport
  Feedback Bus : Inport  Port=2
  1-K_TD : Gain  Gain=1-PitchDampingTrust
  1/ElevatorPower : Gain  Gain=1/ElevatorPower
  "1/ElevatorPower  " : Gain  Gain=1/ElevatorPower
  1st Order Reference Model : Subsystem
  Bus Selector : BusSelector  OutputSignals=Pitch_Euler_rad,Roll_Euler_rad,apMode,DynamicPressure_Pa,PitchRate_Body_radps,V_mps,zAccel_Body_mps2
  Cm/Alpha Estimation : Subsystem
  Compare To Constant : simulink/Logic and Bit Operations/Compare To Constant  relop=<=  const=2  OutDataTypeStr=boolean
  Compare To Constant1 : simulink/Logic and Bit Operations/Compare To Constant  relop===  const=11  OutDataTypeStr=uint8
  Dimensional Elevator Power : Subsystem
  Discrete-Time Integrator1 : DiscreteIntegrator  IntegratorMethod=Integration: Backward Euler  ExternalReset=level  InitialConditionSource=external  SampleTime=-1  LimitOutput=on  UpperSaturationLimit=ElevatorMax  LowerSaturationLimit=-ElevatorMax  ICPrevOutput=DiscIntNeverNeededParam  ICPrevScaledInput=DiscIntNeverNeededParam
  Divide : Product  Inputs=/*
  DynamicPLimit : Subsystem
  Elevator Ramp Logic : Subsystem
  Gain : Gain  Gain=180/pi
  Gain1 : Gain  Gain=-1
  Gain2 : Gain  Gain=pi/180
  Gain3 : Gain  Gain=-1
  KI_Pitch : Gain  Gain=PitchRateErrorInt2Accel
  K_TD : Gain  Gain=PitchDampingTrust
  K_TS : Gain  Gain=PitchStiffnessTrust
  Kp_Pitch : Gain  Gain=PitchRateError2Accel
  LPF Elevator : Subsystem
  Manual Switch : ManualSwitch  CurrentSetting=0
  Manual Switch1 : ManualSwitch  CurrentSetting=0
  NOT : Logic  Operator=NOT  IconShape=distinctive  AllPortsSameDT=off  OutDataTypeStr=boolean
  NOT1 : Logic  Operator=NOT  IconShape=distinctive  AllPortsSameDT=off  OutDataTypeStr=boolean
  OR : Logic  Operator=OR  IconShape=distinctive  AllPortsSameDT=off  OutDataTypeStr=boolean
  Pitch Moment Caused By Damping : Subsystem
  Rad2Deg : Gain  Gain=180/pi
  Reference Frame Conversion and Pitch Rate Limit Determination : Subsystem
  Saturation : Saturate  UpperLimit=ElevatorMax  LowerLimit=-ElevatorMax
  Sum : Sum  Inputs=|+-
  Sum1 : Sum  Inputs=|+--+
  Sum2 : Sum  Inputs=|++
  Sum3 : Sum  Inputs=++|
  Switch : Switch  Criteria=u2 > Threshold
  TASLimit : Subsystem
  Terminator{1..4} (4 alike) : Terminator
  Triggered Subsystem : Subsystem  TreatAsAtomicUnit=on
  Unit Delay : UnitDelay  SampleTime=-1
  constant : Constant  Value=ElevatorTrim  VectorParams1D=off
  resetCondition : Subsystem
  resetVal : Subsystem
  Elevator_Deg : Outport
  tag scope: PicElevatorOut=global, Sim_PitchCmd=global, Sim_PitchRateCmd=global
  wires:
  Compare To Constant1/1 -> OR/2
  OR/1 -> Triggered Subsystem/Trigger, NOT/1
  Compare To Constant/1 -> OR/1
  Rad2Deg/1 -> Terminator1/1  "Sim.PitchCmd"
  resetCondition/1(reset) -> Discrete-Time Integrator1/2
  Bus Selector/6 -> Reference Frame Conversion and Pitch Rate Limit Determination/4(V), TASLimit/2(<V_mps>)  "<V_mps>"
  TASLimit/1(Out1) -> Pitch Moment Caused By Damping/2(TAS)
  Bus Selector/4 -> DynamicPLimit/2(DynamicPressure_Pa)  "<DynamicPressure_Pa>"
  DynamicPLimit/1(Out1) -> Cm/Alpha Estimation/2(Q), Reference Frame Conversion and Pitch Rate Limit Determination/5(Q), Dimensional Elevator Power/1(Dynamic Pressure (Avoid Small Value))
  [Pic_AP_Mode] -> Compare To Constant1/1, Compare To Constant/1
  NOT/1 -> Switch/2
  Switch/1 -> LPF Elevator/1(Input)
  Triggered Subsystem/1(Out1) -> [Elevator_Offset]  "ElevatorOffset"
  Unit Delay/1 -> Triggered Subsystem/1(In1)
  Saturation/1 -> Unit Delay/1, Elevator_Deg/1, Manual Switch1/2  "elevOut"
  [Elevator_Offset] -> Sum1/4
  Reference Frame Conversion and Pitch Rate Limit Determination/3("Scalar ") -> 1st Order Reference Model/3("Scalar ")
  Reference Frame Conversion and Pitch Rate Limit Determination/5("PitchRateLimit_Max ") -> 1st Order Reference Model/5("PitchRateLimit_Max ")
  Sum2/1 -> Pitch Moment Caused By Damping/1(PitchRate_Body)  "Sim.Damp_TrustMix"
  1/ElevatorPower/1 -> Sum1/2, Gain1/1
  Gain2/1 -> Manual Switch/1  "REF.pitchRateCmd"
  Manual Switch/1 -> Sum/1, 1-K_TD/1
  [REFpitchRateCmd] -> Gain2/1  "REF.pitchRateCmdDps"
  Pitch Moment Caused By Damping/1(DAMP) -> 1/ElevatorPower/1
  constant/1 -> Terminator4/1  "Sim.PitchTrim"
  Discrete-Time Integrator1/1 -> Sum3/1  "Sim.KI_Pitch"
  Kp_Pitch/1 -> Sum3/2  "Sim.Kp_Pitch"
  Sum3/1 -> Sum1/1
  Divide/1 -> KI_Pitch/1, Kp_Pitch/1
  KI_Pitch/1 -> Discrete-Time Integrator1/1
  Bus Selector/3 -> 1st Order Reference Model/7(apMode), TASLimit/1(apMode), DynamicPLimit/1(apMode)  "<apMode>"
  Gain/1 -> [Sim_PitchRateCmd]  "Sim.pitchRateCmd"
  Gain1/1 -> Terminator2/1  "Sim.PitchDamp"
  Gain3/1 -> Terminator3/1  "Sim.PitchStiffness"
  "1/ElevatorPower  "/1 -> Sum1/3, Gain3/1
  Sum1/1 -> Switch/1
  Bus Selector/7 -> Cm/Alpha Estimation/1(zAccel_Body)  "<zAccel_Body_mps2>"
  Bus Selector/5 -> 1st Order Reference Model/8(PitchRate_Body), Sum/2, K_TD/1  "<PitchRate_Body_radps>"
  Bus Selector/2 -> Reference Frame Conversion and Pitch Rate Limit Determination/3(Roll_Euler)  "<Roll_Euler_rad>"
  Bus Selector/1 -> Reference Frame Conversion and Pitch Rate Limit Determination/2(Pitch_Euler)  "<Pitch_Euler_rad>"
  Feedback Bus/1 -> Bus Selector/1
  Reference Frame Conversion and Pitch Rate Limit Determination/6("PitchRateLimit_Min ") -> 1st Order Reference Model/6(" PitchRateLimit_Min ")
  Reference Frame Conversion and Pitch Rate Limit Determination/4(PitchRateCmd_Body) -> 1st Order Reference Model/4("PitchRateCmd_Body ")
  PitchCmd_Euler/1 -> [Sim_PitchCmd], Rad2Deg/1, Reference Frame Conversion and Pitch Rate Limit Determination/1(PitchCmd_Euler)
  Dimensional Elevator Power/1(CP) -> Divide/1
  Reference Frame Conversion and Pitch Rate Limit Determination/2("Pitch_Body ") -> 1st Order Reference Model/2("Pitch_Body ")
  Cm/Alpha Estimation/1(STIFF) -> K_TS/1
  K_TD/1 -> Sum2/2
  1-K_TD/1 -> Sum2/1
  1st Order Reference Model/1(PitchRateCmd_Body) -> Gain/1, Manual Switch/2
  Sum/1 -> Divide/2  "Sim.pitchRateErr"
  Reference Frame Conversion and Pitch Rate Limit Determination/1(PitchCmd_Body) -> 1st Order Reference Model/1(PitchCmd_Body)
  [ApGlobal] -> NOT1/1
  NOT1/1 -> LPF Elevator/2(Reset)
  [pilotPitch] -> LPF Elevator/3(ResetValue)  "rstVal"
  resetVal/1(resetVal) -> Discrete-Time Integrator1/3
  Manual Switch1/1 -> [PicElevatorOut]
  [REF_elevator] -> Manual Switch1/1
  Elevator Ramp Logic/1(Elevator Out) -> Switch/3, Saturation/1
  LPF Elevator/1(Output) -> Elevator Ramp Logic/1(Elevator In)  "elevLPFout"
  [Pic_AP_Mode] -> Elevator Ramp Logic/2(AP Mode)
  K_TS/1 -> "1/ElevatorPower  "/1

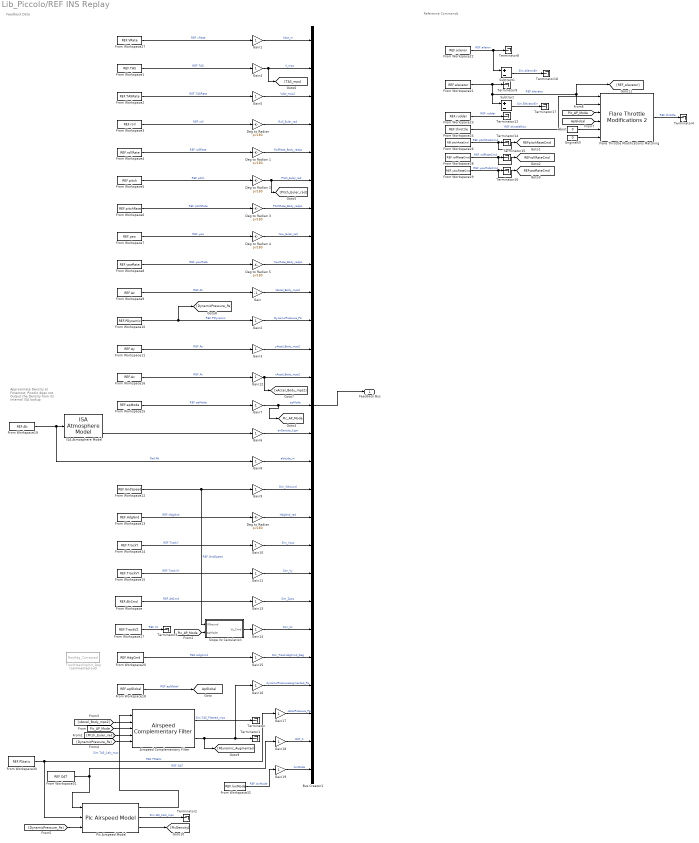
== system Lib_Piccolo/REF INS Replay ==
  note: Feedback Data
  note: Approximate Density at Foremost. Piccolo does not Output the Density from its internal ISA lookup
  note: Reference Commands
  Abort : Constant  Value=0
  Airspeed Complementary Filter : $bdroot/Airspeed Complementary Filter  SystemSampleTime=-1
  Bus Creator1 : BusCreator  Inputs=27
  Deg to Radian : Gain  Gain=pi/180
  Deg to Radian {,1..5} (6 alike) : Gain  Gain=pi/180
  EngineKill : Constant  Value=0
  Flare Throttle Modifications Matching : $bdroot/Throttle Control (Alt Mode)/Flare Throttle Modifications 2  SystemSampleTime=-1
  From Workspace : FromWorkspace  VariableName=REF.AltCmd  SampleTime=0
  From Workspace1 : FromWorkspace  VariableName=REF.TAS  SampleTime=0
  From Workspace10 : FromWorkspace  VariableName=REF.PDynamic  SampleTime=0
  From Workspace11 : FromWorkspace  VariableName=REF.Ay  SampleTime=0
  From Workspace12 : FromWorkspace  VariableName=REF.GndSpeed  SampleTime=0
  From Workspace13 : FromWorkspace  VariableName=REF.HdgGnd  SampleTime=0
  From Workspace14 : FromWorkspace  VariableName=REF.TrackY  SampleTime=0
  From Workspace15 : FromWorkspace  VariableName=REF.TrackVY  SampleTime=0
  From Workspace16 : FromWorkspace  VariableName=REF.Ax  SampleTime=0
  From Workspace17 : FromWorkspace  VariableName=REF.TrackVZ  SampleTime=0
  From Workspace18 : FromWorkspace  VariableName=REF.apGlobal  SampleTime=0
  From Workspace19 : FromWorkspace  VariableName=REF.Alt  SampleTime=0
  From Workspace2 : FromWorkspace  VariableName=REF.TASRate  SampleTime=0
  From Workspace20 : FromWorkspace  VariableName=REF.HdgCmd  SampleTime=0
  From Workspace21 : FromWorkspace  VariableName=REF.elevator  SampleTime=0
  From Workspace22 : FromWorkspace  VariableName=REF.aileron  SampleTime=0
  From Workspace23 : FromWorkspace  VariableName=REF.rudder  SampleTime=0
  From Workspace24 : FromWorkspace  VariableName=REF.throttle  SampleTime=0
  From Workspace25 : FromWorkspace  VariableName=REF.apMode  SampleTime=0
  From Workspace26 : FromWorkspace  VariableName=REF.pitchRateCmd  SampleTime=0
  From Workspace27 : FromWorkspace  VariableName=REF.VRate  SampleTime=0
  From Workspace28 : FromWorkspace  VariableName=REF.rollRateCmd  SampleTime=0
  From Workspace29 : FromWorkspace  VariableName=REF.yawRateCmd  SampleTime=0
  From Workspace3 : FromWorkspace  VariableName=REF.roll  SampleTime=0
  From Workspace30 : FromWorkspace  VariableName=REF.PStatic  SampleTime=0
  From Workspace31 : FromWorkspace  VariableName=REF.OAT  SampleTime=0
  From Workspace32 : FromWorkspace  VariableName=REF.lonMode  SampleTime=0
  From Workspace4 : FromWorkspace  VariableName=REF.rollRate  SampleTime=0
  From Workspace5 : FromWorkspace  VariableName=REF.pitch  SampleTime=0
  From Workspace6 : FromWorkspace  VariableName=REF.pitchRate  SampleTime=0
  From Workspace7 : FromWorkspace  VariableName=REF.yaw  SampleTime=0
  From Workspace8 : FromWorkspace  VariableName=REF.yawRate  SampleTime=0
  From Workspace9 : FromWorkspace  VariableName=REF.Az  SampleTime=0
  Gain : Gain  Gain=-1
  Gain{1..19} (19 alike) : Gain
  ISA Atmosphere Model : aerolibatmos2/ISA Atmosphere Model  custom=off  g=9.80665  gamma=1.4  R=287.0531  L=0.0065  h_trop=11000  h_strat=20000  rho0=1.225  P0=101325  T0=288.15  h0=0
      settings: SourceProductName=Aerospace Blockset
  Pic Airspeed Model : $bdroot/Pic Airspeed Model  correction=1
  Slope Vz Calculation : Subsystem
  Subtract : Sum  Inputs=+-
  Subtract1 : Sum  Inputs=+-
  Terminator{,1..4,8..9,12,14..18} (13 alike) : Terminator
  TrackHeadingInit_Deg : Constant  Commented=on  Value=RwyHdg_Corrected
  Feedback Bus : Outport
  tag scope: ApGlobal=global, Pic_AP_Mode=global, REFpitchRateCmd=global, REFrollRateCmd=global, REFyawRateCmd=global
  wires:
  Deg to Radian 2/1 -> [Pitch_Euler_rad], Bus Creator1/6  "Pitch_Euler_rad"
  Deg to Radian 3/1 -> Bus Creator1/7  "PitchRate_Body_radps"
  Gain/1 -> Bus Creator1/10  "zAccel_Body_mps2"
  Deg to Radian 5/1 -> Bus Creator1/9  "YawRate_Body_radps"
  Deg to Radian 4/1 -> Bus Creator1/8  "Yaw_Euler_rad"
  Bus Creator1/1 -> Feedback Bus/1
  Gain3/1 -> Bus Creator1/12  "yAccel_Body_mps2"
  Gain1/1 -> Bus Creator1/1  "hdot_m"
  Gain4/1 -> [TAS_mps], Bus Creator1/2  "V_mps"
  Gain5/1 -> Bus Creator1/3  "Vdot_mps2"
  "Deg to Radian "/1 -> Bus Creator1/4  "Roll_Euler_rad"
  Deg to Radian 1/1 -> Bus Creator1/5  "RollRate_Body_radps"
  Gain6/1 -> Bus Creator1/15  "airDensity_kgm"
  From Workspace27/1 -> Gain1/1  "REF.vRate"
  From Workspace2/1 -> Gain5/1  "REF.TASRate"
  From Workspace3/1 -> "Deg to Radian "/1  "REF.roll"
  From Workspace4/1 -> Deg to Radian 1/1  "REF.rollRate"
  From Workspace5/1 -> Deg to Radian 2/1  "REF.pitch"
  From Workspace6/1 -> Deg to Radian 3/1  "REF.pitchRate"
  From Workspace7/1 -> Deg to Radian 4/1  "REF.yaw"
  From Workspace8/1 -> Deg to Radian 5/1  "REF.yawRate"
  From Workspace9/1 -> Gain/1  "REF.Az"
  From Workspace10/1 -> [DynamicPressure_Pa], Gain2/1  "REF.PDynamic"
  From Workspace11/1 -> Gain3/1  "REF.Ay"
  ISA Atmosphere Model/4 -> Gain6/1
  From Workspace19/1 -> Gain8/1, ISA Atmosphere Model/1  "Ref.Alt"
  Gain7/1 -> [Pic_AP_Mode], Bus Creator1/14  "apMode"
  From Workspace25/1 -> Gain7/1  "REF.apMode"
  Gain8/1 -> Bus Creator1/16  "altitude_m"
  Gain9/1 -> Bus Creator1/17  "Sim_VGround"
  From Workspace12/1 -> Slope Vz Calculation/1(VGround), Gain9/1  "REF.GndSpeed"
  From Workspace13/1 -> Deg to Radian/1  "REF.HdgGnd"
  Deg to Radian/1 -> Bus Creator1/18  "HdgGnd_rad"
  From Workspace1/1 -> Gain4/1  "REF.TAS"
  From Workspace14/1 -> Gain10/1  "REF.TrackY"
  Gain10/1 -> Bus Creator1/19  "Sim_Ypos"
  From Workspace15/1 -> Gain11/1  "REF.TrackVY"
  Gain11/1 -> Bus Creator1/20  "Sim_Vy"
  From Workspace16/1 -> Gain12/1  "REF.Ax"
  Gain12/1 -> [xAccel_Body_mps2], Bus Creator1/13  "xAccel_Body_mps2"
  From Workspace/1 -> Gain13/1  "REF.AltCmd"
  Gain13/1 -> Bus Creator1/21  "Sim_Zpos"
  Gain14/1 -> Bus Creator1/22  "Sim_Vz"
  From Workspace17/1 -> Terminator3/1  "REF.Vz"
  From Workspace18/1 -> [ApGlobal]  "REF.apGlobal"
  Gain15/1 -> Bus Creator1/23  "Sim_TrackHdgCmd_Deg"
  From Workspace20/1 -> Gain15/1  "REF.HdgCmd"
  [Pic_AP_Mode] -> Airspeed Complementary Filter/3
  [Pitch_Euler_rad] -> Airspeed Complementary Filter/4
  [xAccel_Body_mps2] -> Airspeed Complementary Filter/2
  Airspeed Complementary Filter/1 -> Terminator/1  "Sim.TAS_Filtered_mps"
  [DynamicPressure_Pa] -> Airspeed Complementary Filter/5
  Airspeed Complementary Filter/2 -> [Pdynamic_Augmented], Gain16/1, Terminator1/1
  Gain16/1 -> Bus Creator1/24  "dynamicPressureAugmented_Pa"
  Pic Airspeed Model/1 -> Airspeed Complementary Filter/1  "Sim.TAS_Calc_mps"
  Pic Airspeed Model/2 -> Terminator2/1  "Sim.IAS_Calc_mps"
  [DynamicPressure_Pa] -> Pic Airspeed Model/3
  From Workspace30/1 -> Pic Airspeed Model/2, Gain17/1  "REF.PStatic"
  Gain17/1 -> Bus Creator1/25  "staticPressure_Pa"
  From Workspace31/1 -> Pic Airspeed Model/1, Gain18/1  "REF.OAT"
  Gain18/1 -> Bus Creator1/26  "OAT_C"
  Gain2/1 -> Bus Creator1/11  "DynamicPressure_Pa"
  Pic Airspeed Model/3 -> [PicDensity]
  Slope Vz Calculation/1(Vz_Cmd) -> Gain14/1
  [Pic_AP_Mode] -> Slope Vz Calculation/2(apMode)
  From Workspace24/1 -> Flare Throttle Modifications Matching/1  "REF.throttleRaw"
  Abort/1 -> Flare Throttle Modifications Matching/5
  From Workspace26/1 -> [REFpitchRateCmd], Terminator14/1  "REF.pitchRateCmd"
  From Workspace23/1 -> Terminator12/1  "REF.rudder"
  From Workspace29/1 -> [REFyawRateCmd], Terminator16/1  "REF.yawRateCmd"
  Subtract/1 -> Terminator17/1  "Sim.ElevatorErr"
  [Pic_AP_Mode] -> Flare Throttle Modifications Matching/3
  EngineKill/1 -> Flare Throttle Modifications Matching/6
  From Workspace22/1 -> Terminator8/1, Subtract1/1  "REF.aileron"
  Subtract1/1 -> Terminator18/1  "Sim.AileronErr"
  From Workspace21/1 -> Terminator9/1, [REF_elevator], Flare Throttle Modifications Matching/2, Subtract/1  "REF.elevator"
  Flare Throttle Modifications Matching/1 -> Terminator4/1  "REF.throttle"
  From Workspace28/1 -> [REFrollRateCmd], Terminator15/1  "REF.rollRateCmd"
  [ApGlobal] -> Flare Throttle Modifications Matching/4
  From Workspace32/1 -> Gain19/1  "REF.lonMode"
  Gain19/1 -> Bus Creator1/27  "lonMode"

== system Lib_Piccolo/Sliding Window Maximum ==
  note: Insert new element
  note: Remove last element
  note: Define dimensions
      | (initial conditions)
  windowInput : Inport
  IC : InitialCondition  Value=[zeros(N,1)]
  Max : MinMax  Function=max
  Memory : Memory
  Mux : Mux  Inputs=2
  Variable Selector : dspindex/Variable Selector  NumInputs=1  rowsOrCols=Rows  IdxMode=Fixed  Elements=1:N-1  ZerOneIdxMode=One-based  errmode=Clip Index  FillMode=on  FillValues=0
  windowMax : Outport
  wires:
  Memory/1 -> IC/1
  Mux/1 -> Max/1, Memory/1
  windowInput/1 -> Mux/1
  Variable Selector/1 -> Mux/2
  IC/1 -> Variable Selector/1
  Max/1 -> windowMax/1
